simulink model "x2_foc_svpwm"  (R2024b)
settings: Solver=VariableStepAuto  StartTime=0.0  StopTime=0.5  RelTol=1e-3
undefined symbols (not defined in the file or in its folder): DiscIntNeverNeededParam, Tpwm, Ts, vbus
libraries: simulink x1, spspowerguiLib x1
settings Model: Creator=disnox  LastModifiedBy=cd
settings DataIOCC: ReturnWorkspaceOutputs=off
settings DebuggingCC: ParameterPrecisionLossMsg=none
settings RTWCC: GPUComputeCapability=3.5

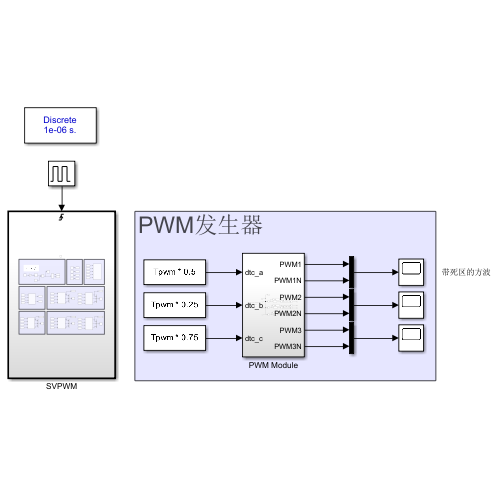
[thumbnail: Simulink's stored preview of the top-level diagram]
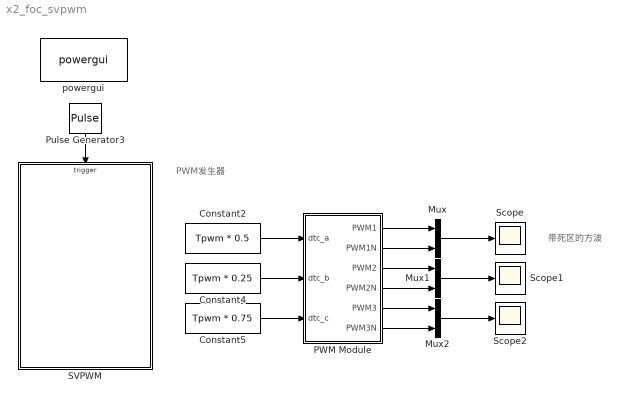
== system x2_foc_svpwm ==
  note: 带死区的方波
  note: PWM发生器
  Constant2 : Constant  Value=Tpwm * 0.5
  Constant4 : Constant  Value=Tpwm * 0.25
  Constant5 : Constant  Value=Tpwm * 0.75
  Mux : Mux  Inputs=2
  Mux1 : Mux  Inputs=2
  Mux2 : Mux  Inputs=2
  PWM Module : Subsystem
  Pulse Generator3 : DiscretePulseGenerator  PulseType=Time based  Period=Ts  PulseWidth=50
  SVPWM : Subsystem
  Scope : Scope
  Scope1 : Scope
  Scope2 : Scope
  powergui : spspowerguiLib/powergui  SimulationMode=Discrete  SampleTime=Ts/100  frequency=60  Iterations=50  frequencyindice=0  Pbase=100e6  ErrMax=1e-4  UnitsV=kV  UnitsW=MW  buscounter=0  FunctionMessages=off  echomessages=off  EnableUseOfTLC=off  CurrentSourceSwitches=off  DisableSnubberDevices=off  DisableRonSwitches=off  DisableVfSwitches=off  DisplayEquations=off  AutomaticDiscreteSolvers=off  SolverType=Tustin/Backward Euler (TBE)  Interpol=off  ExternalGateDelay=off  methode=off  Ts=0  x0status=blocks  SPID=off  SwTol=0  HookPort=off  NonlinearTolerance=1e-4  nMaxIteration=100  ContinueOnMaxIteration=off  RestoreLinks=warning  ResistiveCurrentMeasurement=off  Frange=[0:2:500]  Ylog=off  Xlog=on  ShowGrid=off  save=off  variable=ZData  structure=0  ZoomFFT=off  StartTime=0.0  cycles=1  DisplayStyle=1  fundamental=60  FreqAxis=off  MaxFrequency=1000  frequencyindicesteady=1  RmsSteady=1  display=off
  wires:
  Pulse Generator3/1 -> SVPWM/Trigger
  PWM Module/6(PWM3N) -> Mux2/2
  PWM Module/3(PWM2) -> Mux1/1
  Mux1/1 -> Scope1/1
  Mux2/1 -> Scope2/1
  Mux/1 -> Scope/1
  Constant2/1 -> PWM Module/1(dtc_a)
  PWM Module/1(PWM1) -> Mux/1
  PWM Module/4(PWM2N) -> Mux1/2
  Constant5/1 -> PWM Module/3(dtc_c)
  Constant4/1 -> PWM Module/2(dtc_b)
  PWM Module/5(PWM3) -> Mux2/1
  PWM Module/2(PWM1N) -> Mux/2

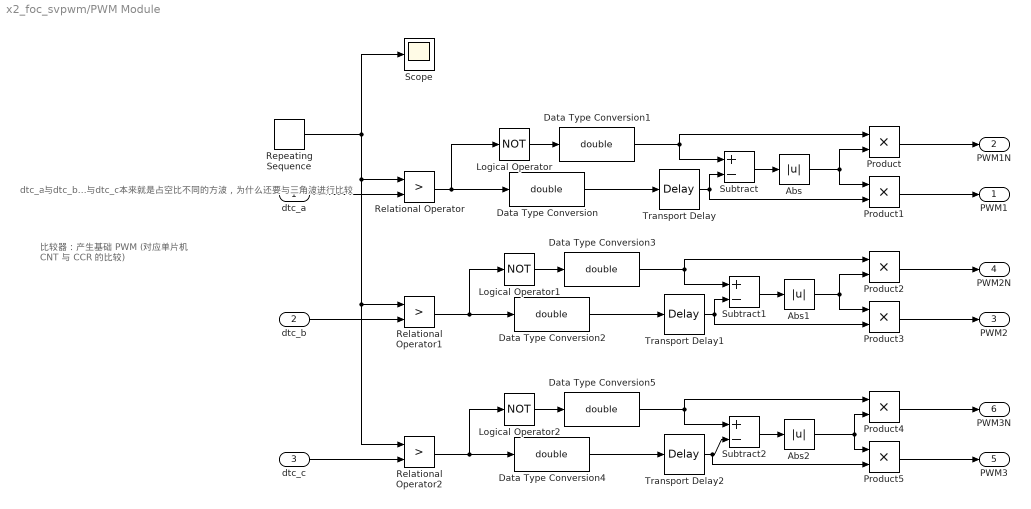
== system x2_foc_svpwm/PWM Module ==
  note: dtc_a与dtc_b与dtc_c本来就是占空比不同的方波，为什么还要与三角波进行比较
  note: 比较器：产生基础 PWM
      | (对应单片机 CNT 与 CCR 的比较)
  dtc_a : Inport
  dtc_b : Inport  Port=2
  dtc_c : Inport  Port=3
  Abs : Abs  SaturateOnIntegerOverflow=off
  Abs1 : Abs  SaturateOnIntegerOverflow=off
  Abs2 : Abs  SaturateOnIntegerOverflow=off
  Data Type Conversion{,1..5} (6 alike) : DataTypeConversion  OutDataTypeStr=double  SaturateOnIntegerOverflow=off  RndMeth=Floor
  Logical Operator : Logic  Operator=NOT  AllPortsSameDT=off  OutDataTypeStr=boolean
  Logical Operator1 : Logic  Operator=NOT  AllPortsSameDT=off  OutDataTypeStr=boolean
  Logical Operator2 : Logic  Operator=NOT  AllPortsSameDT=off  OutDataTypeStr=boolean
  Product{,1..5} (6 alike) : Product
  Relational Operator : RelationalOperator  Operator=>  OutDataTypeStr=boolean  RndMeth=Simplest  InputSameDT=off
  Relational Operator1 : RelationalOperator  Operator=>  OutDataTypeStr=boolean  RndMeth=Simplest  InputSameDT=off
  Relational Operator2 : RelationalOperator  Operator=>  OutDataTypeStr=boolean  RndMeth=Simplest  InputSameDT=off
  Repeating Sequence : simulink/Sources/Repeating Sequence  rep_seq_t=[0 Ts/2 Ts]  rep_seq_y=[0 Tpwm 0]
  Scope : Scope
  Subtract : Sum  Inputs=+-
  Subtract1 : Sum  Inputs=+-
  Subtract2 : Sum  Inputs=+-
  Transport Delay : TransportDelay  DelayTime=168/168e6
  Transport Delay1 : TransportDelay  DelayTime=168/168e6
  Transport Delay2 : TransportDelay  DelayTime=168/168e6
  PWM1 : Outport
  PWM1N : Outport  Port=2
  PWM2 : Outport  Port=3
  PWM2N : Outport  Port=4
  PWM3 : Outport  Port=5
  PWM3N : Outport  Port=6
  wires:
  Product1/1 -> PWM1/1
  Relational Operator1/1 -> Logical Operator1/1, Data Type Conversion2/1
  Logical Operator2/1 -> Data Type Conversion5/1
  Subtract/1 -> Abs/1
  Relational Operator2/1 -> Data Type Conversion4/1, Logical Operator2/1
  Product4/1 -> PWM3N/1
  Data Type Conversion5/1 -> Subtract2/1, Product4/1
  Product2/1 -> PWM2N/1
  Abs1/1 -> Product2/2, Product3/1
  Transport Delay2/1 -> Subtract2/2, Product5/2
  Repeating Sequence/1 -> Scope/1, Relational Operator/1, Relational Operator2/1, Relational Operator1/1
  Data Type Conversion/1 -> Transport Delay/1
  Product/1 -> PWM1N/1
  Product3/1 -> PWM2/1
  Abs2/1 -> Product5/1, Product4/2
  Data Type Conversion2/1 -> Transport Delay1/1
  dtc_a/1 -> Relational Operator/2
  Transport Delay/1 -> Product1/2, Subtract/2
  Subtract1/1 -> Abs1/1
  Data Type Conversion3/1 -> Subtract1/1, Product2/1
  dtc_c/1 -> Relational Operator2/2
  Logical Operator/1 -> Data Type Conversion1/1
  Transport Delay1/1 -> Product3/2, Subtract1/2
  Relational Operator/1 -> Logical Operator/1, Data Type Conversion/1
  Abs/1 -> Product/2, Product1/1
  Product5/1 -> PWM3/1
  Data Type Conversion4/1 -> Transport Delay2/1
  Subtract2/1 -> Abs2/1
  Logical Operator1/1 -> Data Type Conversion3/1
  Data Type Conversion1/1 -> Subtract/1, Product/1
  dtc_b/1 -> Relational Operator1/2

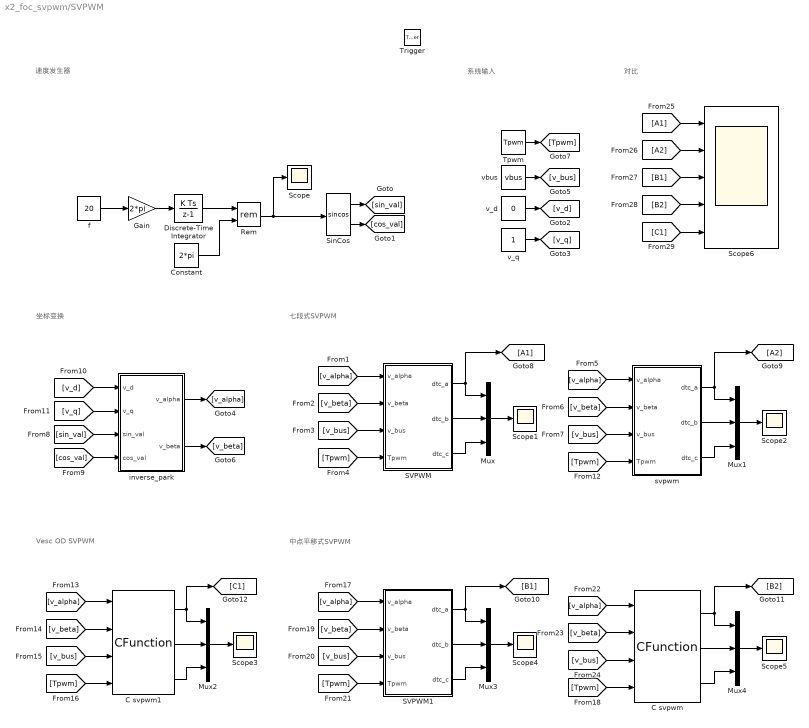
== system x2_foc_svpwm/SVPWM ==
  note: 系统输入
  note: 速度发生器
  note: 坐标变换
  note: 七段式SVPWM
  note: Vesc OD SVPWM
  note: 中点平移式SVPWM
  note: 对比
  Trigger : TriggerPort  VariantControl=(inherit)
  C svpwm : CFunction  OutputCode=|  GenerateCodeAsIs=off  CodegenOutputCode=|  CustomCodeSettingLocation=ModelConfigurationParameters
      | #define ONE_BY_SQRT3			(0.57735026919f)
      | #define TWO_BY_SQRT3			(2.0f * 0.57735026919f)
      | #define SQRT3_BY_2				(0.86602540378f)
      | #define SQRT3 					(1.73205080757f)
      | #define min(x,y) 				(((x)<(y))?(x):(y))
      | #define max(x,y) 				(((x)>(y))?(x):(y))
      | 
      | float v_alpha = valpha/v_bus;
      | float v_beta = vbeta/v_bus;
      | 	
      |   float va = v_alpha;  
      |   float vb = -0.5f * v_alpha + SQRT3_BY_2 * v_beta; 
      |   float vc = -0.5f * v_alpha - SQRT3_BY_2 * v_beta; 
      | 
      | 	float vmax = max(max(va, vb), vc);
      | 	float vmin = min(min(va, vb), vc);
      |   
      |   float vcom = (vmax + vmin) * 0.5f;
      | 	
      | 	dtc_a = ((vcom - va) + 0.5f)*Tpwm;
      | 	dtc_b = ((vcom - vb) + 0.5f)*Tpwm;
      | 	dtc_c = ((vcom - vc) + 0.5f)*Tpwm;
      | #define ONE_BY_SQRT3			(0.57735026919f)
      | #define TWO_BY_SQRT3			(2.0f * 0.57735026919f)
      | #define SQRT3_BY_2				(0.86602540378f)
      | #define SQRT3 					(1.73205080757f)
      | #define min(x,y) 				(((x)<(y))?(x):(y))
      | #define max(x,y) 				(((x)>(y))?(x):(y))
      | 
      | float v_alpha = valpha/v_bus;
      | float v_beta = vbeta/v_bus;
      | 	
      |   float va = v_alpha;  
      |   float vb = -0.5f * v_alpha + SQRT3_BY_2 * v_beta; 
      |   float vc = -0.5f * v_alpha - SQRT3_BY_2 * v_beta; 
      | 
      | 	float vmax = max(max(va, vb), vc);
      | 	float vmin = min(min(va, vb), vc);
      |   
      |   float vcom = (vmax + vmin) * 0.5f;
      | 	
      | 	dtc_a = ((vcom - va) + 0.5f)*Tpwm;
      | 	dtc_b = ((vcom - vb) + 0.5f)*Tpwm;
      | 	dtc_c = ((vcom - vc) + 0.5f)*Tpwm;
  C svpwm1 : CFunction  OutputCode=|  GenerateCodeAsIs=off  CodegenOutputCode=|  CustomCodeSettingLocation=ModelConfigurationParameters
      | #define ONE_BY_SQRT3			(0.57735026919f)
      | #define TWO_BY_SQRT3			(2.0f * 0.57735026919f)
      | #define SQRT3_BY_2				(0.86602540378f)
      | 
      | float tA;
      | float tB;
      | float tC;
      | 
      | int Sextant;
      | 
      | float v_alpha = valpha/(v_bus*0.67f);
      | float v_beta = vbeta/(v_bus*0.67f);
      | 
      | if (v_beta >= 0.0f) {
      | 		if (v_alpha >= 0.0f) {
      | 				//quadrant I
      | 				if (ONE_BY_SQRT3 * v_beta > v_alpha) Sextant = 2; //sextant v2-v3
      | 				else Sextant = 1; //sextant v1-v2
      | 
      | 		} else {
      | 				//quadrant II
      | 				if (-ONE_BY_SQRT3 * v_beta > v_alpha) Sextant = 3; //sextant v3-v4
      | 				else Sextant = 2; //sextant v2-v3
      | 		}
      | } else {
      | 		if (v_alpha >= 0.0f) {
      | 				//quadrant IV
      | 				if (-ONE_BY_SQRT3 * v_beta > v_alpha) Sextant = 5; //sextant v5-v6
      | 				else Sextant = 6; //sextant v6-v1
      | 		} else {
      | 				//quadrant III
      | 				if (ONE_BY_SQRT3 * v_beta > v_alpha) Sextant = 4; //sextant v4-v5
      | 				else Sextant = 5; //sextant v5-v6
      | 		}
      | }
      | 
      | switch (Sextant) {
      | 		// sextant v1-v2
      | case 1:
      | 		{
      | 				// Vector on-times
      | 				float t1 = v_alpha - ONE_BY_SQRT3 * v_beta;
      | 				float t2 = TWO_BY_SQRT3 * v_beta;
      | 
      | 				// PWM timings
      | 				tA = (1.0f - t1 - t2) * 0.5f;
      | 				tB = tA + t1;
      | 				tC = tB + t2;
      | 		}
      | 		break;
      | 
      | 		// sextant v2-v3
      | case 2:
      | 		{
      | 				// Vector on-times
      | 				float t2 = v_alpha + ONE_BY_SQRT3 * v_beta;
      | 				float t3 = -v_alpha + ONE_BY_SQRT3 * v_beta;
      | 
      | 				// PWM timings
      | 				tB = (1.0f - t2 - t3) * 0.5f;
      | 				tA = tB + t3;
      | 				tC = tA + t2;
      | 		}
      | 		break;
      | 
      | 		// sextant v3-v4
      | case 3:
      | 		{
      | 				// Vector on-times
      | 				float t3 = TWO_BY_SQRT3 * v_beta;
      | 				float t4 = -v_alpha - ONE_BY_SQRT3 * v_beta;
      | 
      | 				// PWM timings
      | 				tB = (1.0f - t3 - t4) * 0.5f;
      | 				tC = tB + t3;
      | 				tA = tC + t4;
      | 		}
      | 		break;
      | 
      | 		// sextant v4-v5
      | case 4:
      | 		{
      | 				// Vector on-times
      | 				float t4 = -v_alpha + ONE_BY_SQRT3 * v_beta;
      | 				float t5 = -TWO_BY_SQRT3 * v_beta;
      | 
      | 				// PWM timings
      | 				tC = (1.0f - t4 - t5) * 0.5f;
      | 				tB = tC + t5;
      | 				tA = tB + t4;
      | 		}
      | 		break;
      | 
      | 		// sextant v5-v6
      | case 5:
      | 		{
      | 				// Vector on-times
      | 				float t5 = -v_alpha - ONE_BY_SQRT3 * v_beta;
      | 				float t6 = v_alpha - ONE_BY_SQRT3 * v_beta;
      | 
      | 				// PWM timings
      | 				tC = (1.0f - t5 - t6) * 0.5f;
      | 				tA = tC + t5;
      | 				tB = tA + t6;
      | 		}
      | 		break;
      | 
      | 		// sextant v6-v1
      | case 6:
      | 		{
      | 				// Vector on-times
      | 				float t6 = -TWO_BY_SQRT3 * v_beta;
      | 				float t1 = v_alpha + ONE_BY_SQRT3 * v_beta;
      | 
      | 				// PWM timings
      | 				tA = (1.0f - t6 - t1) * 0.5f;
      | 				tC = tA + t1;
      | 				tB = tC + t6;
      | 		}
      | 		break;
      | }
      | 
      | // if any of the results becomes NaN, result_valid will evaluate to false
      | int result_valid =
      | 		tA >= 0.0f && tA <= 1.0f
      | 		&& tB >= 0.0f && tB <= 1.0f
      | 		&& tC >= 0.0f && tC <= 1.0f;
      | 
      | dtc_a = Tpwm*tA;
      | dtc_b = Tpwm*tB;
      | dtc_c = Tpwm*tC;
      | #define ONE_BY_SQRT3			(0.57735026919f)
      | #define TWO_BY_SQRT3			(2.0f * 0.57735026919f)
      | #define SQRT3_BY_2				(0.86602540378f)
      | 
      | float tA;
      | float tB;
      | float tC;
      | 
      | int Sextant;
      | 
      | float v_alpha = valpha/(v_bus*0.67f);
      | float v_beta = vbeta/(v_bus*0.67f);
      | 
      | if (v_beta >= 0.0f) {
      | 		if (v_alpha >= 0.0f) {
      | 				//quadrant I
      | 				if (ONE_BY_SQRT3 * v_beta > v_alpha) Sextant = 2; //sextant v2-v3
      | 				else Sextant = 1; //sextant v1-v2
      | 
      | 		} else {
      | 				//quadrant II
      | 				if (-ONE_BY_SQRT3 * v_beta > v_alpha) Sextant = 3; //sextant v3-v4
      | 				else Sextant = 2; //sextant v2-v3
      | 		}
      | } else {
      | 		if (v_alpha >= 0.0f) {
      | 				//quadrant IV
      | 				if (-ONE_BY_SQRT3 * v_beta > v_alpha) Sextant = 5; //sextant v5-v6
      | 				else Sextant = 6; //sextant v6-v1
      | 		} else {
      | 				//quadrant III
      | 				if (ONE_BY_SQRT3 * v_beta > v_alpha) Sextant = 4; //sextant v4-v5
      | 				else Sextant = 5; //sextant v5-v6
      | 		}
      | }
      | 
      | switch (Sextant) {
      | 		// sextant v1-v2
      | case 1:
      | 		{
      | 				// Vector on-times
      | 				float t1 = v_alpha - ONE_BY_SQRT3 * v_beta;
      | 				float t2 = TWO_BY_SQRT3 * v_beta;
      | 
      | 				// PWM timings
      | 				tA = (1.0f - t1 - t2) * 0.5f;
      | 				tB = tA + t1;
      | 				tC = tB + t2;
      | 		}
      | 		break;
      | 
      | 		// sextant v2-v3
      | case 2:
      | 		{
      | 				// Vector on-times
      | 				float t2 = v_alpha + ONE_BY_SQRT3 * v_beta;
      | 				float t3 = -v_alpha + ONE_BY_SQRT3 * v_beta;
      | 
      | 				// PWM timings
      | 				tB = (1.0f - t2 - t3) * 0.5f;
      | 				tA = tB + t3;
      | 				tC = tA + t2;
      | 		}
      | 		break;
      | 
      | 		// sextant v3-v4
      | case 3:
      | 		{
      | 				// Vector on-times
      | 				float t3 = TWO_BY_SQRT3 * v_beta;
      | 				float t4 = -v_alpha - ONE_BY_SQRT3 * v_beta;
      | 
      | 				// PWM timings
      | 				tB = (1.0f - t3 - t4) * 0.5f;
      | 				tC = tB + t3;
      | 				tA = tC + t4;
      | 		}
      | 		break;
      | 
      | 		// sextant v4-v5
      | case 4:
      | 		{
      | 				// Vector on-times
      | 				float t4 = -v_alpha + ONE_BY_SQRT3 * v_beta;
      | 				float t5 = -TWO_BY_SQRT3 * v_beta;
      | 
      | 				// PWM timings
      | 				tC = (1.0f - t4 - t5) * 0.5f;
      | 				tB = tC + t5;
      | 				tA = tB + t4;
      | 		}
      | 		break;
      | 
      | 		// sextant v5-v6
      | case 5:
      | 		{
      | 				// Vector on-times
      | 				float t5 = -v_alpha - ONE_BY_SQRT3 * v_beta;
      | 				float t6 = v_alpha - ONE_BY_SQRT3 * v_beta;
      | 
      | 				// PWM timings
      | 				tC = (1.0f - t5 - t6) * 0.5f;
      | 				tA = tC + t5;
      | 				tB = tA + t6;
      | 		}
      | 		break;
      | 
      | 		// sextant v6-v1
      | case 6:
      | 		{
      | 				// Vector on-times
      | 				float t6 = -TWO_BY_SQRT3 * v_beta;
      | 				float t1 = v_alpha + ONE_BY_SQRT3 * v_beta;
      | 
      | 				// PWM timings
      | 				tA = (1.0f - t6 - t1) * 0.5f;
      | 				tC = tA + t1;
      | 				tB = tC + t6;
      | 		}
      | 		break;
      | }
      | 
      | // if any of the results becomes NaN, result_valid will evaluate to false
      | int result_valid =
      | 		tA >= 0.0f && tA <= 1.0f
      | 		&& tB >= 0.0f && tB <= 1.0f
      | 		&& tC >= 0.0f && tC <= 1.0f;
      | 
      | dtc_a = Tpwm*tA;
      | dtc_b = Tpwm*tB;
      | dtc_c = Tpwm*tC;
  Constant : Constant  Value=2*pi
  Discrete-Time Integrator : DiscreteIntegrator  SampleTime=-1  ICPrevOutput=DiscIntNeverNeededParam  ICPrevScaledInput=DiscIntNeverNeededParam
  Gain : Gain  Gain=2*pi
  Mux{,1..4} (5 alike) : Mux  Inputs=3
  Rem : Math  Operator=rem
  SVPWM : Subsystem  TreatAsAtomicUnit=on
      settings: RTWSystemCode=Nonreusable function  RTWFcnNameOpts=Use subsystem name
  SVPWM1 : Subsystem  TreatAsAtomicUnit=on
      settings: RTWSystemCode=Nonreusable function  RTWFcnNameOpts=Use subsystem name
  Scope{,1..5} (6 alike) : Scope
  Scope6 : Scope  NumInputPorts=5
  SinCos : Trigonometry  Operator=sincos
  Tpwm : Constant  Value=Tpwm
  f : Constant  Value=20
  inverse_park : Subsystem  TreatAsAtomicUnit=on
      settings: RTWSystemCode=Nonreusable function  RTWFcnNameOpts=Use subsystem name
  svpwm : MATLAB Function  TreatAsAtomicUnit=on
  v_d : Constant  Value=0
  v_q : Constant
  vbus : Constant  Value=vbus
  wires:
  SinCos/1 -> [sin_val]
  SinCos/2 -> [cos_val]
  v_q/1 -> [v_q]
  v_d/1 -> [v_d]
  [cos_val] -> inverse_park/4(cos_val)
  [v_d] -> inverse_park/1(v_d)
  [v_q] -> inverse_park/2(v_q)
  [sin_val] -> inverse_park/3(sin_val)
  Constant/1 -> Rem/2
  f/1 -> Gain/1
  Gain/1 -> Discrete-Time Integrator/1
  Discrete-Time Integrator/1 -> Rem/1
  Rem/1 -> SinCos/1, Scope/1
  inverse_park/1(v_alpha) -> [v_alpha]
  inverse_park/2(v_beta) -> [v_beta]
  [v_alpha] -> SVPWM/1(v_alpha)
  [v_beta] -> SVPWM/2(v_beta)
  SVPWM/2(dtc_b) -> Mux/2
  SVPWM/1(dtc_a) -> [A1], Mux/1
  SVPWM/3(dtc_c) -> Mux/3
  Mux/1 -> Scope1/1
  vbus/1 -> [v_bus]
  [v_bus] -> SVPWM/3(v_bus)
  Tpwm/1 -> [Tpwm]
  [Tpwm] -> SVPWM/4(Tpwm)
  Mux1/1 -> Scope2/1
  svpwm/3(dtc_c) -> Mux1/3
  [Tpwm] -> svpwm/4(Tpwm)
  [v_bus] -> svpwm/3(v_bus)
  svpwm/2(dtc_b) -> Mux1/2
  svpwm/1(dtc_a) -> [A2], Mux1/1
  [v_alpha] -> svpwm/1(v_alpha)
  [v_beta] -> svpwm/2(v_beta)
  Mux2/1 -> Scope3/1
  C svpwm1/3 -> Mux2/3
  [Tpwm] -> C svpwm1/4
  [v_bus] -> C svpwm1/3
  C svpwm1/2 -> Mux2/2
  C svpwm1/1 -> [C1], Mux2/1
  [v_alpha] -> C svpwm1/1
  [v_beta] -> C svpwm1/2
  Mux3/1 -> Scope4/1
  [v_beta] -> SVPWM1/2(v_beta)
  [v_alpha] -> SVPWM1/1(v_alpha)
  Mux4/1 -> Scope5/1
  C svpwm/1 -> [B2], Mux4/1
  [v_bus] -> C svpwm/3
  C svpwm/3 -> Mux4/3
  [v_beta] -> C svpwm/2
  C svpwm/2 -> Mux4/2
  [Tpwm] -> C svpwm/4
  [Tpwm] -> SVPWM1/4(Tpwm)
  [v_bus] -> SVPWM1/3(v_bus)
  [v_alpha] -> C svpwm/1
  SVPWM1/3(dtc_c) -> Mux3/3
  SVPWM1/2(dtc_b) -> Mux3/2
  SVPWM1/1(dtc_a) -> [B1], Mux3/1
  [A1] -> Scope6/1
  [A2] -> Scope6/2
  [B1] -> Scope6/3
  [B2] -> Scope6/4
  [C1] -> Scope6/5

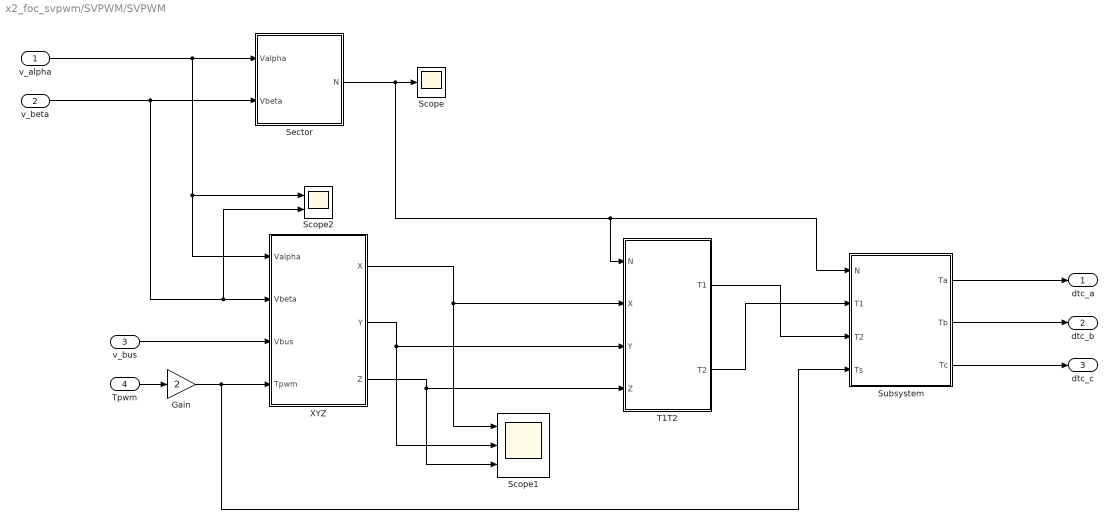
== system x2_foc_svpwm/SVPWM/SVPWM ==
  v_alpha : Inport
  v_beta : Inport  Port=2
  v_bus : Inport  Port=3
  Tpwm : Inport  Port=4
  Gain : Gain  Gain=2
  Scope : Scope
  Scope1 : Scope  NumInputPorts=3
  Scope2 : Scope  NumInputPorts=2
  Sector : Subsystem
  Subsystem : Subsystem
  T1T2 : Subsystem
  XYZ : Subsystem
  dtc_a : Outport
  dtc_b : Outport  Port=2
  dtc_c : Outport  Port=3
  wires:
  v_alpha/1 -> Scope2/1, XYZ/1(Valpha), Sector/1(Valpha)
  v_beta/1 -> Scope2/2, XYZ/2(Vbeta), Sector/2(Vbeta)
  Sector/1(N) -> Subsystem/1(N), T1T2/1(N), Scope/1
  v_bus/1 -> XYZ/3(Vbus)
  XYZ/1(X) -> Scope1/1, T1T2/2(X)
  XYZ/2(Y) -> Scope1/2, T1T2/3(Y)
  XYZ/3(Z) -> T1T2/4(Z), Scope1/3
  T1T2/1(T1) -> Subsystem/3(T2)
  T1T2/2(T2) -> Subsystem/2(T1)
  Subsystem/1(Ta) -> dtc_a/1
  Subsystem/2(Tb) -> dtc_b/1
  Subsystem/3(Tc) -> dtc_c/1
  Tpwm/1 -> Gain/1
  Gain/1 -> XYZ/4(Tpwm), Subsystem/4(Ts)

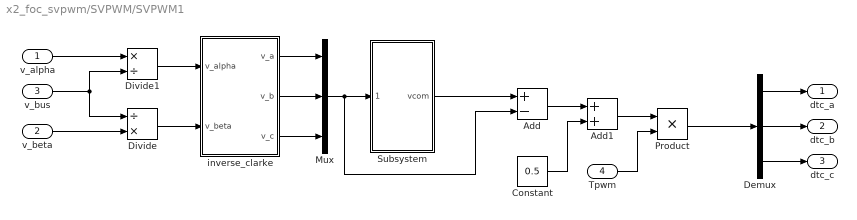
== system x2_foc_svpwm/SVPWM/SVPWM1 ==
  v_alpha : Inport
  v_beta : Inport  Port=2
  v_bus : Inport  Port=3
  Tpwm : Inport  Port=4
  Add : Sum  Inputs=+-
  Add1 : Sum
  Constant : Constant  Value=0.5
  Demux : Demux  Outputs=3
  Divide : Product  Inputs=/*
  Divide1 : Product  Inputs=*/
  Mux : Mux  Inputs=3
  Product : Product
  Subsystem : Subsystem
  inverse_clarke : Subsystem  TreatAsAtomicUnit=on
      settings: RTWSystemCode=Nonreusable function  RTWFcnNameOpts=Use subsystem name
  dtc_a : Outport
  dtc_b : Outport  Port=2
  dtc_c : Outport  Port=3
  wires:
  Demux/1 -> dtc_a/1
  Demux/2 -> dtc_b/1
  Demux/3 -> dtc_c/1
  inverse_clarke/2(v_b) -> Mux/2
  inverse_clarke/1(v_a) -> Mux/1
  inverse_clarke/3(v_c) -> Mux/3
  Mux/1 -> Subsystem/1(v_abc), Add/2
  Subsystem/1(vcom) -> Add/1
  Add/1 -> Add1/1
  Constant/1 -> Add1/2
  Add1/1 -> Product/1
  Product/1 -> Demux/1
  Tpwm/1 -> Product/2
  Divide/1 -> inverse_clarke/2(v_beta)
  Divide1/1 -> inverse_clarke/1(v_alpha)
  v_alpha/1 -> Divide1/1
  v_beta/1 -> Divide/2
  v_bus/1 -> Divide/1, Divide1/2

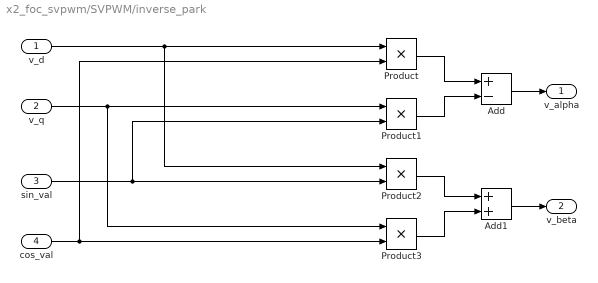
== system x2_foc_svpwm/SVPWM/inverse_park ==
  v_d : Inport
  v_q : Inport  Port=2
  sin_val : Inport  Port=3
  cos_val : Inport  Port=4
  Add : Sum  Inputs=+-
  Add1 : Sum  AccumDataTypeStr=double
  Product{,1..3} (4 alike) : Product
  v_alpha : Outport
  v_beta : Outport  Port=2
  wires:
  v_d/1 -> Product2/1, Product/1
  cos_val/1 -> Product3/2, Product/2
  Product/1 -> Add/1
  Product1/1 -> Add/2
  v_q/1 -> Product1/1, Product3/1
  sin_val/1 -> Product2/2, Product1/2
  Add/1 -> v_alpha/1
  Product2/1 -> Add1/1
  Product3/1 -> Add1/2
  Add1/1 -> v_beta/1

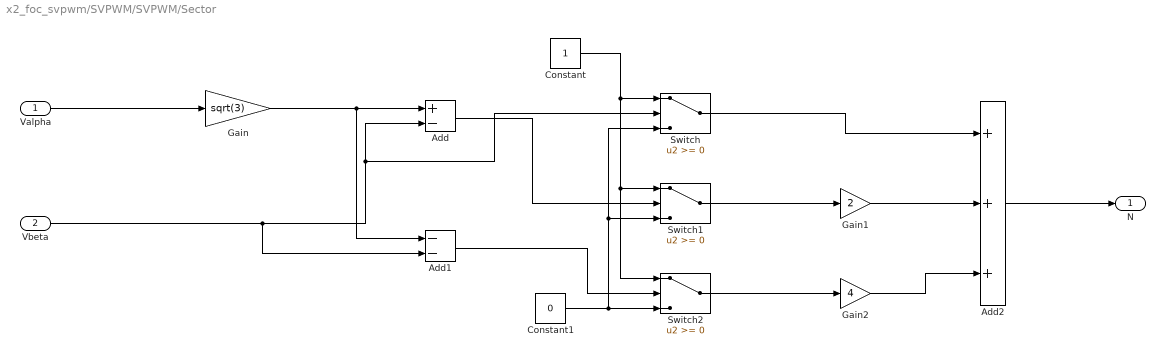
== system x2_foc_svpwm/SVPWM/SVPWM/Sector ==
  Valpha : Inport
  Vbeta : Inport  Port=2
  Add : Sum  Inputs=+-  OutDataTypeStr=single  AccumDataTypeStr=single
  Add1 : Sum  Inputs=--  OutDataTypeStr=single  AccumDataTypeStr=single
  Add2 : Sum  Inputs=+++
  Constant : Constant  OutDataTypeStr=single
  Constant1 : Constant  Value=0  OutDataTypeStr=single
  Gain : Gain  Gain=sqrt(3)
  Gain1 : Gain  Gain=2
  Gain2 : Gain  Gain=4
  Switch : Switch  SaturateOnIntegerOverflow=off  InputSameDT=off
  Switch1 : Switch  SaturateOnIntegerOverflow=off  InputSameDT=off
  Switch2 : Switch  SaturateOnIntegerOverflow=off  InputSameDT=off
  N : Outport
  wires:
  Valpha/1 -> Gain/1
  Gain/1 -> Add1/1, Add/1
  Vbeta/1 -> Add1/2, Switch/2, Add/2
  Constant1/1 -> Switch/3, Switch1/3, Switch2/3
  Constant/1 -> Switch2/1, Switch1/1, Switch/1
  Add1/1 -> Switch2/2
  Add/1 -> Switch1/2
  Switch1/1 -> Gain1/1
  Switch2/1 -> Gain2/1
  Gain2/1 -> Add2/3
  Gain1/1 -> Add2/2
  Switch/1 -> Add2/1
  Add2/1 -> N/1

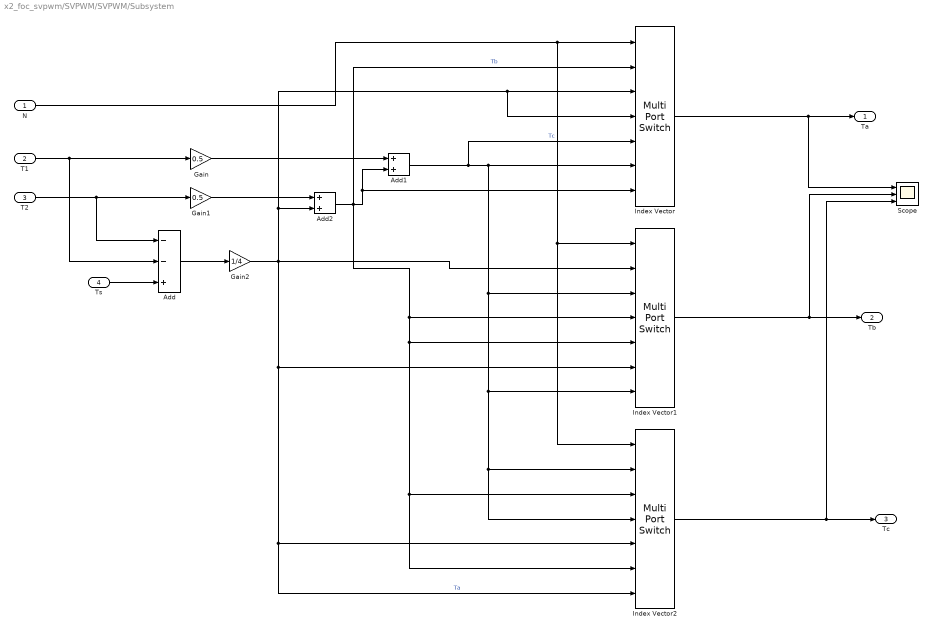
== system x2_foc_svpwm/SVPWM/SVPWM/Subsystem ==
  N : Inport
  T1 : Inport  Port=2
  T2 : Inport  Port=3
  Ts : Inport  Port=4
  Add : Sum  Inputs=--+
  Add1 : Sum
  Add2 : Sum
  Gain : Gain  Gain=0.5
  Gain1 : Gain  Gain=0.5
  Gain2 : Gain  Gain=1/4
  Index Vector : MultiPortSwitch  Inputs=6  SaturateOnIntegerOverflow=off  InputSameDT=off
  Index Vector1 : MultiPortSwitch  Inputs=6  SaturateOnIntegerOverflow=off  InputSameDT=off
  Index Vector2 : MultiPortSwitch  Inputs=6  SaturateOnIntegerOverflow=off  InputSameDT=off
  Scope : Scope  NumInputPorts=3
  Ta : Outport
  Tb : Outport  Port=2
  Tc : Outport  Port=3
  wires:
  T1/1 -> Add/2, Gain/1
  T2/1 -> Add/1, Gain1/1
  Add/1 -> Gain2/1
  Gain1/1 -> Add2/1
  Gain2/1 -> Index Vector1/2, Index Vector/4, Index Vector/3, Add2/2, Index Vector2/7, Index Vector2/5, Index Vector1/6  "Ta"
  Gain/1 -> Add1/1
  Add2/1 -> Index Vector2/6, Index Vector2/3, Index Vector1/5, Index Vector1/4, Index Vector/7, Add1/2, Index Vector/2  "Tb"
  Add1/1 -> Index Vector/5, Index Vector/6, Index Vector1/3, Index Vector1/7, Index Vector2/4, Index Vector2/2  "Tc"
  N/1 -> Index Vector2/1, Index Vector1/1, Index Vector/1
  Index Vector/1 -> Scope/1, Ta/1
  Index Vector1/1 -> Scope/2, Tb/1
  Index Vector2/1 -> Tc/1, Scope/3
  Ts/1 -> Add/3

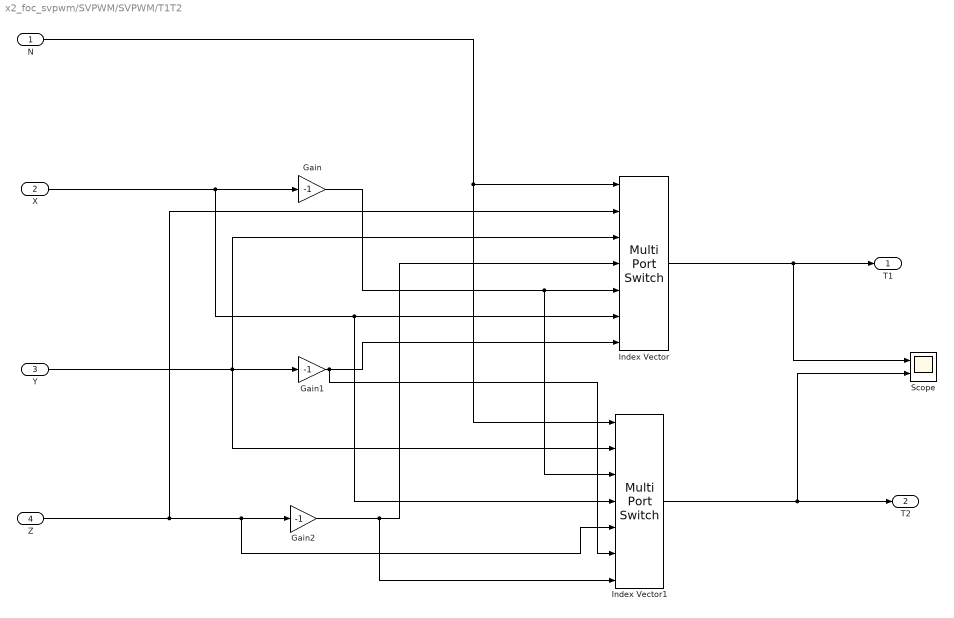
== system x2_foc_svpwm/SVPWM/SVPWM/T1T2 ==
  N : Inport
  X : Inport  Port=2
  Y : Inport  Port=3
  Z : Inport  Port=4
  Gain : Gain  Gain=-1
  Gain1 : Gain  Gain=-1
  Gain2 : Gain  Gain=-1
  Index Vector : MultiPortSwitch  Inputs=6  SaturateOnIntegerOverflow=off  InputSameDT=off
  Index Vector1 : MultiPortSwitch  Inputs=6  SaturateOnIntegerOverflow=off  InputSameDT=off
  Scope : Scope  NumInputPorts=2
  T1 : Outport
  T2 : Outport  Port=2
  wires:
  X/1 -> Index Vector1/4, Index Vector/6, Gain/1
  Y/1 -> Index Vector1/2, Index Vector/3, Gain1/1
  Z/1 -> Index Vector/2, Index Vector1/5, Gain2/1
  Index Vector/1 -> Scope/1, T1/1
  Index Vector1/1 -> Scope/2, T2/1
  N/1 -> Index Vector1/1, Index Vector/1
  Gain2/1 -> Index Vector1/7, Index Vector/4
  Gain/1 -> Index Vector1/3, Index Vector/5
  Gain1/1 -> Index Vector1/6, Index Vector/7

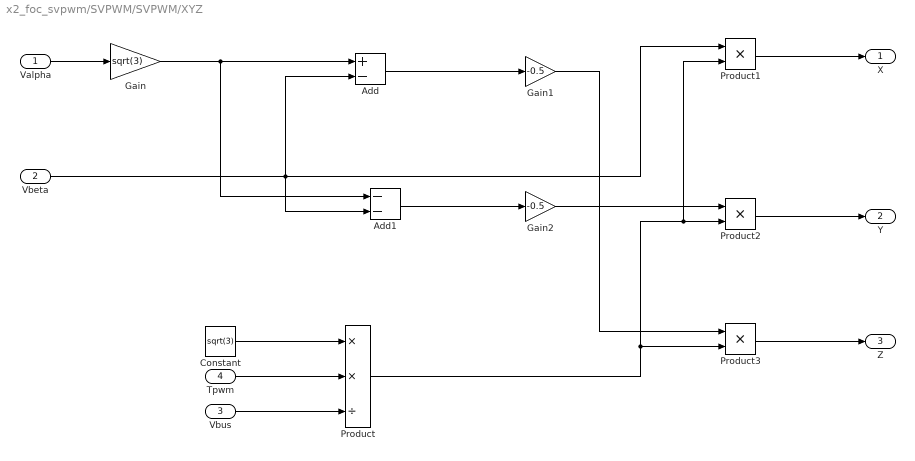
== system x2_foc_svpwm/SVPWM/SVPWM/XYZ ==
  Valpha : Inport
  Vbeta : Inport  Port=2
  Vbus : Inport  Port=3
  Tpwm : Inport  Port=4
  Add : Sum  Inputs=+-
  Add1 : Sum  Inputs=--
  Constant : Constant  Value=sqrt(3)
  Gain : Gain  Gain=sqrt(3)
  Gain1 : Gain  Gain=-0.5
  Gain2 : Gain  Gain=-0.5
  Product : Product  Inputs=**/
  Product1 : Product
  Product2 : Product
  Product3 : Product
  X : Outport
  Y : Outport  Port=2
  Z : Outport  Port=3
  wires:
  Valpha/1 -> Gain/1
  Vbeta/1 -> Product1/1, Add/2, Add1/2
  Gain/1 -> Add1/1, Add/1
  Add/1 -> Gain1/1
  Add1/1 -> Gain2/1
  Constant/1 -> Product/1
  Tpwm/1 -> Product/2
  Vbus/1 -> Product/3
  Gain1/1 -> Product3/1
  Gain2/1 -> Product2/1
  Product/1 -> Product3/2, Product1/2, Product2/2
  Product1/1 -> X/1
  Product2/1 -> Y/1
  Product3/1 -> Z/1

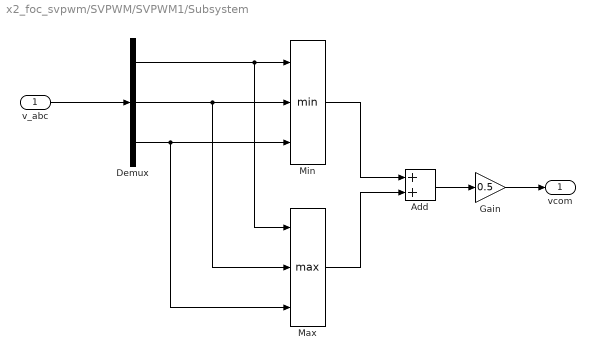
== system x2_foc_svpwm/SVPWM/SVPWM1/Subsystem ==
  v_abc : Inport
  Add : Sum
  Demux : Demux  Outputs=3
  Gain : Gain  Gain=0.5
  Max : MinMax  Function=max  Inputs=3
  Min : MinMax  Inputs=3
  vcom : Outport
  wires:
  Min/1 -> Add/1
  Max/1 -> Add/2
  Add/1 -> Gain/1
  Gain/1 -> vcom/1
  Demux/1 -> Max/1, Min/1
  Demux/2 -> Max/2, Min/2
  Demux/3 -> Max/3, Min/3
  v_abc/1 -> Demux/1

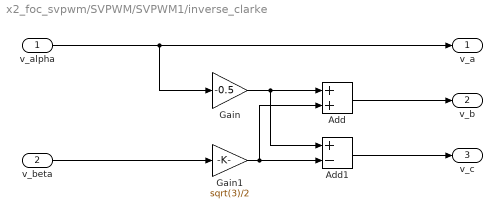
== system x2_foc_svpwm/SVPWM/SVPWM1/inverse_clarke ==
  v_alpha : Inport
  v_beta : Inport  Port=2
  Add : Sum
  Add1 : Sum  Inputs=+-
  Gain : Gain  Gain=-0.5
  Gain1 : Gain  Gain=sqrt(3)/2
  v_a : Outport
  v_b : Outport  Port=2
  v_c : Outport  Port=3
  wires:
  v_alpha/1 -> Gain/1, v_a/1
  Gain/1 -> Add1/1, Add/1
  v_beta/1 -> Gain1/1
  Gain1/1 -> Add/2, Add1/2
  Add/1 -> v_b/1
  Add1/1 -> v_c/1

== matlab function x2_foc_svpwm/SVPWM/svpwm ==
  data: dtc_a output; v_alpha input; v_beta input; v_bus input; Tpwm input; dtc_b output; dtc_c output
function [dtc_a,dtc_b,dtc_c] = svpwm(v_alpha, v_beta, v_bus, Tpwm)

Ta=double(0);
Tb=double(0);

N=0;
Tpwm = 2*Tpwm;
A = v_beta;
B = sqrt(3)/2*v_alpha-0.5*v_beta;
C = -sqrt(3)/2*v_alpha-0.5*v_beta;

if(A>0)
    N=N+1;
end
if(B>0)
    N=N+2;
end
if(C>0)
    N=N+4;
end

X=(sqrt(3)*Tpwm)/v_bus*v_beta;
Y=(sqrt(3)*Tpwm)/v_bus*((sqrt(3)/2)*v_alpha+0.5*v_beta);
Z=(sqrt(3)*Tpwm)/v_bus*(-(sqrt(3)/2)*v_alpha+0.5*v_beta);

if(N==3)  %{扇区1 %}
    Ta=-Z;
    Tb=X;
end
if(N==1)  %{扇区2%}
    Ta=Z;
    Tb=Y;
end
if(N==5)  %{扇区3%}
    Ta=X;
    Tb=-Y;
end
if(N==4)  %{扇区4%}
    Ta=-X;
    Tb=Z;
end
if(N==6)  %{扇区5%}
    Ta=-Y;
    Tb=-Z;
end
if(N==2)  %{扇区6%}
    Ta=Y;
    Tb=-X;
end
Tsum = Ta+Tb;
if(Tsum>Tpwm)  %过调制
    Ta=Tpwm*Ta/Tsum;
    Tb=Tpwm*Tb/Tsum;
end

dtc_a=double(0);
dtc_b=double(0);
dtc_c=double(0);

Value1=(Tpwm-Ta-Tb)/4.0;
Value2=Value1+Ta/2.0;
Value3=Value2+Tb/2.0;

switch(N)
    case 3  %{扇区1 %}
        dtc_a=Value1;
        dtc_b=Value2;
        dtc_c=Value3;

    case 1  %{扇区2%}
        dtc_a=Value2;
        dtc_b=Value1;
        dtc_c=Value3;

    case 5  %{扇区3%}
        dtc_a=Value3;
        dtc_b=Value1;
        dtc_c=Value2;

    case 4  %{扇区4%}
        dtc_a=Value3;
        dtc_b=Value2;
        dtc_c=Value1;

    case 6  %{扇区5%}
        dtc_a=Value2;
        dtc_b=Value3;
        dtc_c=Value1;

    case 2  %{扇区6%}
        dtc_a=Value1;
        dtc_b=Value3;
        dtc_c=Value2;
end
